simulink model "dcsim_rt"  (R2026a)
settings: Solver=FixedStepDiscrete  StopTime=T_record  FixedStep=1e-06
values from neighbouring files (symbols this model uses):
  cfg = get_param([mdl '/' name], 'MATLABFunctionConfiguration')    [build_dcsim_shelf.m]
  pv = [800 132000 0.0242424242424 8e-05 0.0005 5e-06 0.005 0.008 640 0.0001 20 288.75 ... (36 elements, 36x1)]    [dcsim_rt_hil_data.mat]    (also in dcsim_rt_hil_demo.m = dcsim_rt_pv(shared, c); dcsim_rt_pv.m = [shared.V_ref; shared.P_rated; shared.R_droop; shared.tau_c;; hil_quickstart.m = evalin('base', 'pv'); rt_hil_check.m = dcsim_rt_pv(shared, c))
  y0 = [797.942200076 84.8842468493 797.517778842 0 84.8842468493 797.263126102 67675.0799999 0.000903675421673 1320 50 0]    [dcsim_rt_hil_data.mat]    (also in dcsim_rt_hil_demo.m = dcsim_rt_hil_y0(pv_y0, P0, dt); dcsim_rt_hil_y0.m = y; dcsim_rt_init.m = [ic.v_c; ic.i_L; ic.v_C; ic.i_f; ic.i_Lin; ic.v_Cin; ic.P_cm; run_hil_handover.m = dcsim_rt_hil_y0(pv_y0, 0.5 * shared.P_rated, dt))
undefined symbols (not defined in the file or in its folder): t_event
Description:
  | dcsim_rt build 2026-10-10 (MODEL.md 0.4.4 + breaker element)
settings Model: Creator=USER  LastModifiedBy=USER

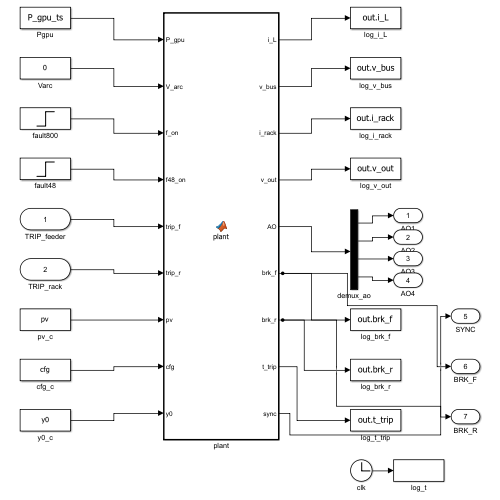
[thumbnail: Simulink's stored preview of the top-level diagram]
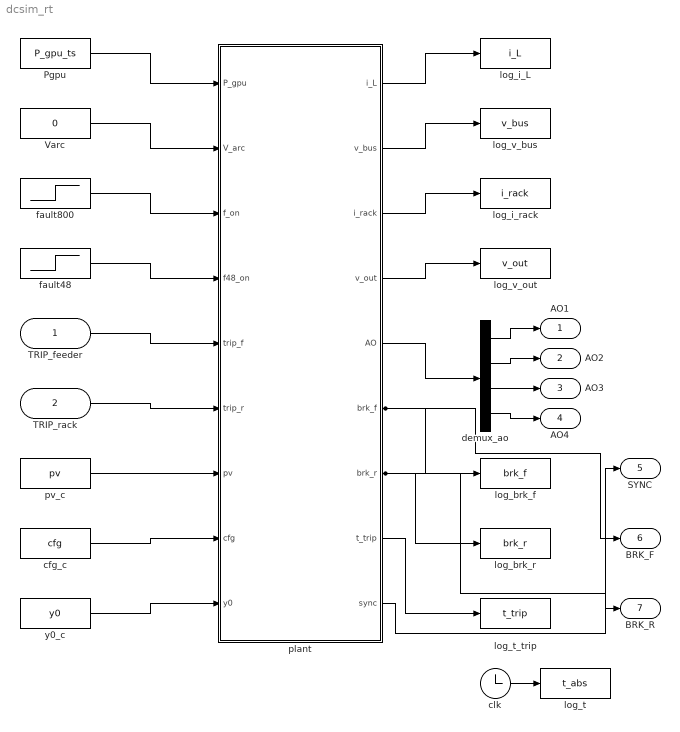
== system dcsim_rt ==
  TRIP_feeder : Inport  SampleTime=1e-06
  TRIP_rack : Inport  Port=2  SampleTime=1e-06
  Pgpu : FromWorkspace  VariableName=P_gpu_ts  OutputAfterFinalValue=Holding final value
  Varc : Constant  Value=0
  cfg_c : Constant  Value=cfg
  clk : Clock
  demux_ao : Demux
  fault48 : Step  Time=t_event  FinalValue=f48_on  SampleTime=1e-06
  fault800 : Step  Time=t_event  FinalValue=f800_on  SampleTime=1e-06
  log_brk_f : ToWorkspace  VariableName=brk_f  SampleTime=-1
  log_brk_r : ToWorkspace  VariableName=brk_r  SampleTime=-1
  log_i_L : ToWorkspace  VariableName=i_L  SampleTime=-1
  log_i_rack : ToWorkspace  VariableName=i_rack  SampleTime=-1
  log_t : ToWorkspace  VariableName=t_abs  SampleTime=-1
  log_t_trip : ToWorkspace  VariableName=t_trip  SampleTime=-1
  log_v_bus : ToWorkspace  VariableName=v_bus  SampleTime=-1
  log_v_out : ToWorkspace  VariableName=v_out  SampleTime=-1
  plant : MATLAB Function  TreatAsAtomicUnit=on
  pv_c : Constant  Value=pv
  y0_c : Constant  Value=y0
  AO1 : Outport
  AO2 : Outport  Port=2
  AO3 : Outport  Port=3
  AO4 : Outport  Port=4
  SYNC : Outport  Port=5
  BRK_F : Outport  Port=6
  BRK_R : Outport  Port=7
  wires:
  Pgpu/1 -> plant/1(P_gpu)
  Varc/1 -> plant/2(V_arc)
  fault800/1 -> plant/3(f_on)
  fault48/1 -> plant/4(f48_on)
  TRIP_feeder/1 -> plant/5(trip_f)
  TRIP_rack/1 -> plant/6(trip_r)
  pv_c/1 -> plant/7(pv)
  cfg_c/1 -> plant/8(cfg)
  y0_c/1 -> plant/9(y0)
  plant/1(i_L) -> log_i_L/1
  plant/2(v_bus) -> log_v_bus/1
  plant/3(i_rack) -> log_i_rack/1
  plant/4(v_out) -> log_v_out/1
  plant/5(AO) -> demux_ao/1
  demux_ao/1 -> AO1/1
  demux_ao/2 -> AO2/1
  demux_ao/3 -> AO3/1
  demux_ao/4 -> AO4/1
  plant/6(brk_f) -> log_brk_f/1, BRK_F/1
  plant/7(brk_r) -> log_brk_r/1, BRK_R/1
  plant/8(t_trip) -> log_t_trip/1
  plant/9(sync) -> SYNC/1
  clk/1 -> log_t/1

== matlab function dcsim_rt/plant ==
  data: P_gpu input; i_L output; V_arc input; f_on input; f48_on input; trip_f input; trip_r input; pv input; cfg input; y0 input; v_bus output; i_rack output; v_out output; AO output; brk_f output; brk_r output; t_trip output; sync output
function [i_L, v_bus, i_rack, v_out, AO, brk_f, brk_r, t_trip, sync] = plant(P_gpu, V_arc, f_on, f48_on, trip_f, trip_r, pv, cfg, y0)
%#codegen
% MODEL.md v0.4.4 plant, one fixed step per call (dcsim_rt_step), plus the breaker element and HIL scaling.
persistent y st brkf brkr tmr_f tmr_r t_now t_inc t_tf t_tr
if isempty(y)
    y = y0; st = [1;1;0;0]; brkf = 1.0; brkr = 1.0; tmr_f = 0.0; tmr_r = 0.0; t_now = 0.0; t_inc = -1.0; t_tf = -1.0; t_tr = -1.0;
end
dt = cfg(1); qs = cfg(2); dly = cfg(3); utol = cfg(4);
sync = 0.0;
if t_inc < 0.0 && (f_on > 0.5 || f48_on > 0.5), t_inc = t_now; sync = 1.0; end
if trip_f > 0.5
    tmr_f = tmr_f + dt;
    if tmr_f >= dly, if brkf > 0.5, t_tf = t_now; end, brkf = 0.0; end
else
    tmr_f = 0.0;
end
if trip_r > 0.5
    tmr_r = tmr_r + dt;
    if tmr_r >= dly, if brkr > 0.5, t_tr = t_now; end, brkr = 0.0; end
else
    tmr_r = 0.0;
end
[y, st, o] = dcsim_rt_step(y, st, pv, dt, P_gpu, V_arc, f_on, f48_on, brkf, brkr, qs, utol);
i_L = o(2); v_bus = o(3); i_rack = o(15); v_out = o(10);
I_r = pv(2) / pv(1); I48 = pv(2) / pv(25);
AO = [10.0 * i_L / (2.64 * I_r); 10.0 * v_bus / (1.45 * pv(1)); 10.0 * i_rack / (16.5 * I48); 10.0 * v_out / (1.45 * pv(25))];
AO = min(max(AO, 0.0), 10.0);
brk_f = brkf; brk_r = brkr;
t_trip = [t_tf; t_tr];
if t_inc >= 0.0, t_trip = t_trip - t_inc; end
t_now = t_now + dt;
end
